simulink model "ecu_boostm"  (R2026a)
settings: Solver=FixedStepDiscrete  StopTime=10  FixedStep=0.001  SampleTimeConstraint=STIndependent
Description:
  | Boost rail warnings. Source of truth for firmware/gen/ecu_boostm.
settings Model: Creator=jj1001000  LastModifiedBy=jj1001000
settings OptimizationCC: DefaultUnderspecifiedDataType=single
settings DebuggingCC: ParameterPrecisionLossMsg=none
settings HardwareCC: ProdLargestAtomicInteger=Long  ProdLargestAtomicFloat=Double  ProdHWDeviceType=ARM Compatible->ARM Cortex-M
settings RTWCC: SystemTargetFile=ert.tlc  GenCodeOnly=on  Description=Embedded Coder
settings ERTTargetCC: UtilityFuncGeneration=Shared location  IncludeMdlTerminateFcn=off  CodeInterfacePackaging=Reusable function  SupportNonFinite=off

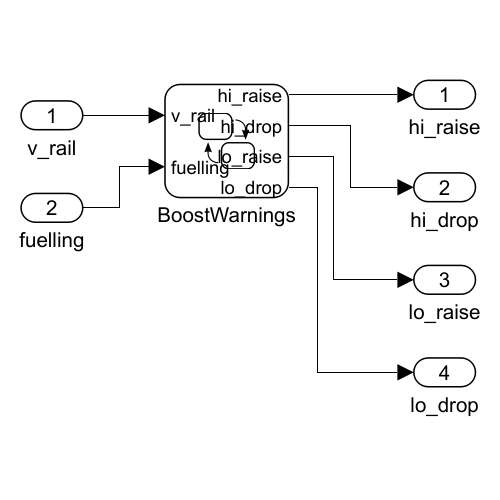
[thumbnail: Simulink's stored preview of the top-level diagram]
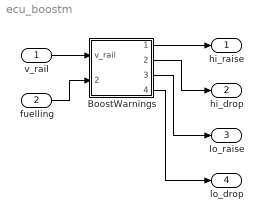
== system ecu_boostm ==
  v_rail : Inport  OutDataTypeStr=single
  fuelling : Inport  Port=2  OutDataTypeStr=uint8
  BoostWarnings : Stateflow chart  TreatAsAtomicUnit=on
  hi_raise : Outport  OutDataTypeStr=uint8
  hi_drop : Outport  Port=2  OutDataTypeStr=uint8
  lo_raise : Outport  Port=3  OutDataTypeStr=uint8
  lo_drop : Outport  Port=4  OutDataTypeStr=uint8
  wires:
  v_rail/1 -> BoostWarnings/1(v_rail)
  fuelling/1 -> BoostWarnings/2(fuelling)
  BoostWarnings/4(lo_drop) -> lo_drop/1
  BoostWarnings/3(lo_raise) -> lo_raise/1
  BoostWarnings/2(hi_drop) -> hi_drop/1
  BoostWarnings/1(hi_raise) -> hi_raise/1

== stateflow chart ecu_boostm/BoostWarnings ==
  settings: updateMethod=DISCRETE  executeAtInitialization=1
  state HIGH [parallel]
    settings: executionOrder=1
    state CLEARING
      entry: hi_raise = uint8(0); hi_drop = uint8(0);
      during: nh = nh + 1;
    state SETTING
      entry: hi_raise = uint8(0); hi_drop = uint8(0);
      during: nh = nh + 1;
    state CLEAR
      entry: hi_raise = uint8(0); hi_drop = uint8(1);
    state SET
      entry: hi_raise = uint8(1); hi_drop = uint8(0);
    (default) -> HIGH.CLEARING : {nh = uint16(0); hi_raise = uint8(0); hi_drop = uint8(0);}
    HIGH.CLEARING -> HIGH.SETTING [order 1] : [v_rail > single(104)]{nh = uint16(1);}
    HIGH.SETTING -> HIGH.CLEARING [order 1] : [~(v_rail > single(104))]{nh = uint16(1);}
    HIGH.CLEARING -> HIGH.CLEAR [order 2] : [nh + 1 >= uint16(2000)]
    HIGH.SET -> HIGH.CLEARING : [~(v_rail > single(104))]{nh = uint16(1);}
    HIGH.CLEAR -> HIGH.SETTING : [v_rail > single(104)]{nh = uint16(1);}
    HIGH.SETTING -> HIGH.SET [order 2] : [nh + 1 >= uint16(2000)]
  state LOW [parallel]
    settings: executionOrder=2
    state CLEARING
      entry: lo_raise = uint8(0); lo_drop = uint8(0);
      during: nl = nl + 1;
    state SETTING
      entry: lo_raise = uint8(0); lo_drop = uint8(0);
      during: nl = nl + 1;
    state CLEAR
      entry: lo_raise = uint8(0); lo_drop = uint8(1);
    state SET
      entry: lo_raise = uint8(1); lo_drop = uint8(0);
    (default) -> LOW.CLEARING : {nl = uint16(0); lo_raise = uint8(0); lo_drop = uint8(0);}
    LOW.CLEARING -> LOW.SETTING [order 1] : [fuelling ~= 0 && v_rail > single(0) && v_rail < single(80)]{nl = uint16(1);}
    LOW.SETTING -> LOW.CLEARING [order 1] : [~(fuelling ~= 0 && v_rail > single(0) && v_rail < single(80))]{nl = uint16(1);}
    LOW.CLEARING -> LOW.CLEAR [order 2] : [nl + 1 >= uint16(500)]
    LOW.SET -> LOW.CLEARING : [~(fuelling ~= 0 && v_rail > single(0) && v_rail < single(80))]{nl = uint16(1);}
    LOW.CLEAR -> LOW.SETTING : [fuelling ~= 0 && v_rail > single(0) && v_rail < single(80)]{nl = uint16(1);}
    LOW.SETTING -> LOW.SET [order 2] : [nl + 1 >= uint16(500)]
  data: v_rail input single; fuelling input uint8; hi_raise output uint8; hi_drop output uint8; lo_raise output uint8; lo_drop output uint8; nh local uint16; nl local uint16
